simulink model "lab1"  (R2022b)
settings: Solver=VariableStepAuto  StartTime=0.0  StopTime=0.35  FixedStep=0.002  RelTol=1e-3  EnableMultiTasking=on
model workspace (MAT data in the model file):
  J = 3.2284e-06
  K = 0.0274
  Kd = 0.0025
  Ki = 1.68
  Kp = 0.461
  L = 2.75e-06
  R = 4
  b = 3.5077e-06
settings Model: ExtModeTrigDuration=10000  Creator=phama10  LastModifiedBy=phama10
settings SolverCC: AlgebraicLoopSolver=TrustRegion  PositivePriorityOrder=on
settings DataIOCC: ReturnWorkspaceOutputs=off
settings DebuggingCC: UnconnectedInputMsg=warning  UnconnectedOutputMsg=warning  UnconnectedLineMsg=warning  SFMachineParentedDataDiag=warning  ArithmeticOperatorsInVariantConditions=warning
settings ModelReferenceCC: EnableRefExpFcnMdlSchedulingChecks=on
settings SFSimCC: SimUseLocalCustomCode=off  CustomCodeUndefinedFunction=UseInterfaceOnly
settings RTWCC: Description=QUARC Win64 Target Using Toolchain  SystemTargetFile=quarc_win64.tlc  TemplateMakefile=quarc_default_tmf  RTWUseLocalCustomCode=off  Toolchain=QUARC win64 | nmake (64-bit Windows)  BuildConfiguration=Faster Runs
settings CodeAppCC: StateflowObjectComments=on
settings STFCustomTargetCC: TargetLangStandard=C99 (ISO)  ConcurrentExecutionCompliant=on  GRTInterface=on  UseToolchainInfoCompliant=on  SystemTargetFile=quarc_win64.tlc
settings GRTTargetCC: ParMdlRefBuildCompliant=off  CompOptLevelCompliant=off  CombineOutputUpdateFcns=off  MatFileLogging=off  CPPClassGenCompliant=off  GRTInterface=on  ExtMode=on  ExtModeMexFile=quarc_comm
settings ConfigComp: CovMetricSettings=dswe

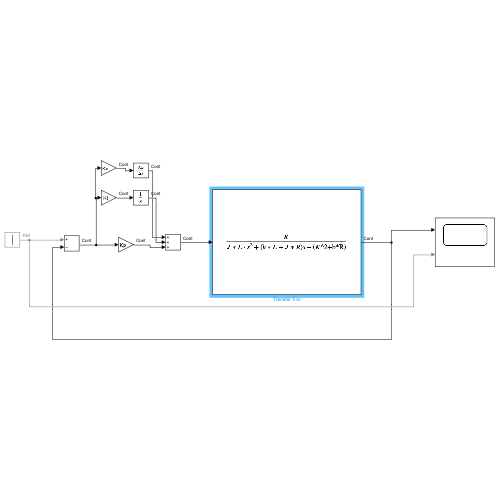
[thumbnail: Simulink's stored preview of the top-level diagram]
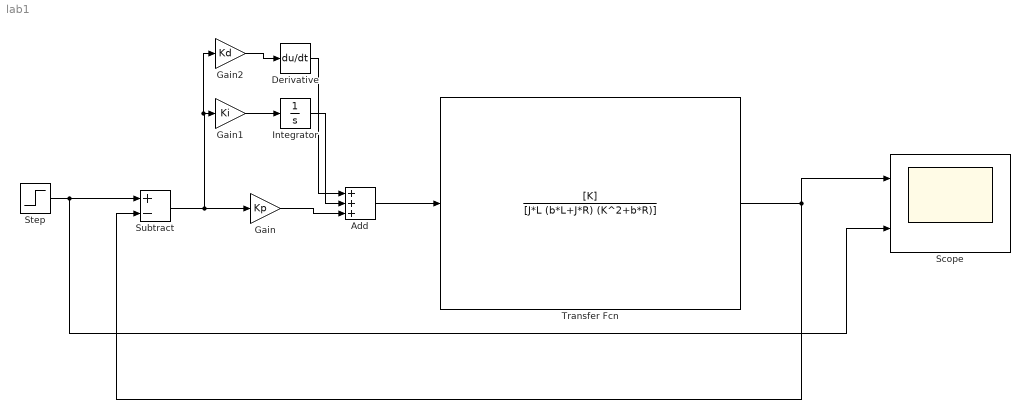
== system lab1 ==
  Add : Sum  Inputs=+++
  Derivative : Derivative
  Gain : Gain  Gain=Kp
  Gain1 : Gain  Gain=Ki
  Gain2 : Gain  Gain=Kd
  Integrator : Integrator
  Scope : Scope  NumInputPorts=2
  Step : Step  Time=0.01  After=60  SampleTime=0
  Subtract : Sum  Inputs=+-
  Transfer Fcn : TransferFcn  Numerator=[K]  Denominator=[J*L (b*L+J*R) (K^2+b*R)]
  wires:
  Step/1 -> Scope/2, Subtract/1
  Transfer Fcn/1 -> Subtract/2, Scope/1
  Gain/1 -> Add/3
  Subtract/1 -> Gain2/1, Gain1/1, Gain/1
  Add/1 -> Transfer Fcn/1
  Gain1/1 -> Integrator/1
  Integrator/1 -> Add/2
  Gain2/1 -> Derivative/1
  Derivative/1 -> Add/1
